simulink model "EMSLEVEL1"  (R2026a)
settings: Solver=FixedStepDiscrete  StopTime=86400  FixedStep=60
InitFcn:
  | params_ems;
  | cap = p.invACDC(p.P_lim);
values from neighbouring files (symbols this model uses):
  p = evalin('base', 'p')    [make_figures.m]    (also in params_ems.m = struct())
undefined symbols (not defined in the file or in its folder): DiscIntNeverNeededParam
settings Model: Creator=Kratos  LastModifiedBy=Kratos

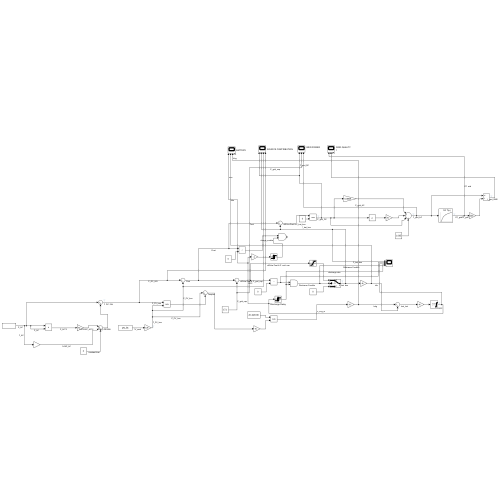
[thumbnail: Simulink's stored preview of the top-level diagram]
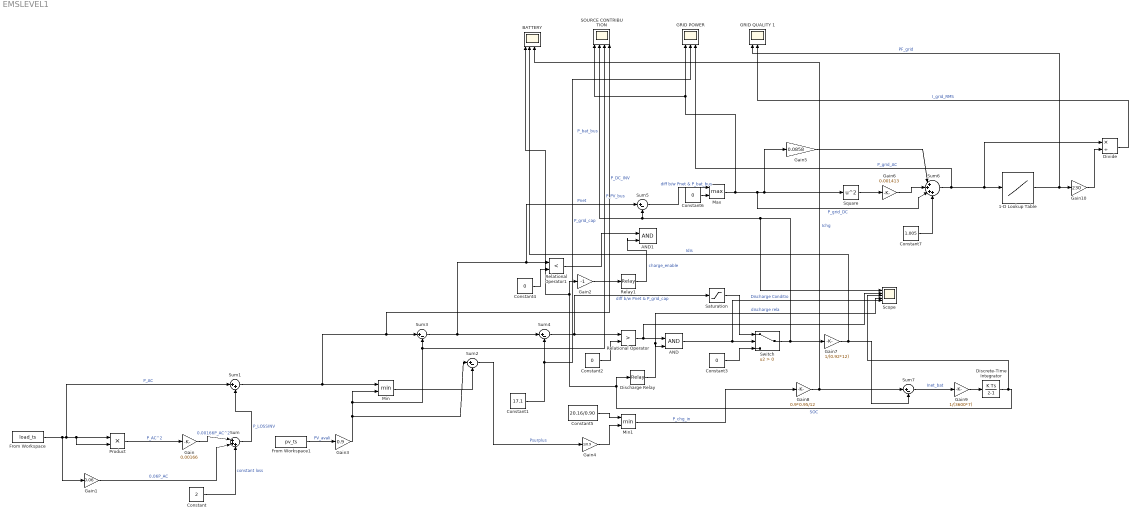
== system EMSLEVEL1 ==
  1-D Lookup Table : Lookup_n-D  NumberOfTableDimensions=1  BreakpointsForDimension1=[3.2 15.1 27.7 41.1 55.2]  Table=[0.308 0.364 0.386 0.399 0.408]  InternalRulePriority=Speed  RndMeth=Simplest
  AND : Logic  IconShape=distinctive  AllPortsSameDT=off  OutDataTypeStr=boolean
  AND1 : Logic  IconShape=distinctive  AllPortsSameDT=off  OutDataTypeStr=boolean
  BATTERY : Scope  NumInputPorts=4
      settings: ActiveDisplayYMinimum=0.046832535784003426  ActiveDisplayYMaximum=1.8408412036240656  DataLoggingVariableName=ScopeData2
  Constant : Constant  Value=2
  Constant1 : Constant  Value=17.1
  Constant{2..4,6} (4 alike) : Constant  Value=0
  Constant5 : Constant  Value=20.16/0.90
  Constant7 : Constant  Value=1.005
  Discharge Relay : Relay  OnSwitchValue=0.43  OffSwitchValue=0.40
  Discrete-Time Integrator : DiscreteIntegrator  InitialCondition=0.9  SampleTime=-1  LimitOutput=on  UpperSaturationLimit=1  LowerSaturationLimit=0  ICPrevOutput=DiscIntNeverNeededParam  ICPrevScaledInput=DiscIntNeverNeededParam
  Divide : Product  Inputs=*/
  From Workspace : FromWorkspace  VariableName=load_ts  SampleTime=60
  From Workspace1 : FromWorkspace  VariableName=pv_ts  SampleTime=60
  "GRID POWER " : Scope  NumInputPorts=3
      settings: ActiveDisplayYMinimum=6.4477565718978767  ActiveDisplayYMaximum=26.985680765987613
  GRID QUALITY 1 : Scope  NumInputPorts=3
      settings: ActiveDisplayYMinimum=-0.12702909452752709  ActiveDisplayYMaximum=0.73391197065675973  DataLoggingVariableName=ScopeData3
  Gain : Gain  Gain=0.00166
  Gain1 : Gain  Gain=0.06
  Gain10 : Gain  Gain=230
  Gain2 : Gain  Gain=-1
  Gain3 : Gain  Gain=0.9
  Gain4 : Gain  Gain=1/0.9
  Gain5 : Gain  Gain=0.0858
  Gain6 : Gain  Gain=0.001413
  Gain7 : Gain  Gain=1/(0.92*12)
  Gain8 : Gain  Gain=0.9*0.95/12
  Gain9 : Gain  Gain=1/(3600*7)
  Max : MinMax  Function=max  Inputs=2
  Min : MinMax  Inputs=2
  Min1 : MinMax  Inputs=2
  Product : Product
  Relational Operator : RelationalOperator  Operator=>  OutDataTypeStr=boolean  RndMeth=Simplest  InputSameDT=off
  Relational Operator1 : RelationalOperator  Operator=<  OutDataTypeStr=boolean  RndMeth=Simplest  InputSameDT=off
  Relay1 : Relay  OnSwitchValue=-0.87  OffSwitchValue=-0.90
  SOURCE CONTRIBUTION : Scope  NumInputPorts=4
      settings: ActiveDisplayYMinimum=28.409856286057689  ActiveDisplayYMaximum=45.225421172870654
  Saturation : Saturate  UpperLimit=30  LowerLimit=0
  Scope : Scope  NumInputPorts=5
      settings: ActiveDisplayYMinimum=-2.8927017969937969  ActiveDisplayYMaximum=27.832680981084884  DataLoggingVariableName=ScopeData4
  Square : Math  Operator=square
  Sum : Sum  Inputs=|+++
  Sum1 : Sum  Inputs=|++
  Sum{2..5,7} (5 alike) : Sum  Inputs=|+-
  Sum6 : Sum  Inputs=|++++
  Switch : Switch  Criteria=u2 > Threshold  SaturateOnIntegerOverflow=off  InputSameDT=off
  wires:
  From Workspace/1 -> Gain1/1, Sum1/1, Product/2, Product/1  "P_AC"
  Product/1 -> Gain/1  "P_AC^2"
  Gain/1 -> Sum/1  "0.00166P_AC^2"
  Gain1/1 -> Sum/2  "0.06P_AC"
  Constant/1 -> Sum/3  "constant loss"
  Sum/1 -> Sum1/2  "P_LOSSINV"
  Sum1/1 -> SOURCE CONTRIBUTION/4, Sum3/1, Min/1  "P_DC_INV"
  From Workspace1/1 -> Gain3/1  "PV_avali"
  Gain3/1 -> SOURCE CONTRIBUTION/3, Sum3/2, Min/2, Sum2/1  "P_PV_bus"
  Min/1 -> Sum2/2
  Sum2/1 -> Gain4/1  "Psurplus"
  Sum3/1 -> Sum5/1, Relational Operator1/1, Sum4/1  "Pnet"
  Gain2/1 -> Relay1/1
  Constant1/1 -> "GRID POWER "/2, Sum4/2  "P_grid_cap"
  Sum4/1 -> Saturation/1, Relational Operator/1  "diff b/w Pnet & P_grid_cap"
  Constant2/1 -> Relational Operator/2
  Relational Operator/1 -> Scope/2, AND/1
  Discharge Relay/1 -> Scope/4, AND/2  "discharge rela"
  AND/1 -> Scope/5, Switch/2  "Discharge Conditio"
  Saturation/1 -> Switch/1
  Constant3/1 -> Switch/3
  Switch/1 -> Scope/1, SOURCE CONTRIBUTION/2, Sum5/2, Gain7/1  "P_bat_bus"
  Constant4/1 -> Relational Operator1/2
  Relational Operator1/1 -> AND1/1
  Relay1/1 -> AND1/2  "charge_enable"
  Constant5/1 -> Min1/1
  Gain4/1 -> Min1/2
  Min1/1 -> Gain8/1  "P_chg_in"
  Sum5/1 -> Max/1  "diff b/w Pnet & P_bat_bus"
  Constant6/1 -> Max/2
  Max/1 -> Sum6/3, Gain5/1, Square/1, SOURCE CONTRIBUTION/1, "GRID POWER "/1  "P_grid_DC"
  Square/1 -> Gain6/1
  Gain5/1 -> Sum6/1
  Gain6/1 -> Sum6/2
  Constant7/1 -> Sum6/4
  Sum6/1 -> Divide/1, 1-D Lookup Table/1, "GRID POWER "/3  "P_grid_AC"
  Gain7/1 -> BATTERY/2, Sum7/2  "Idis"
  Gain8/1 -> Sum7/1, BATTERY/3  "Ichg"
  Sum7/1 -> Gain9/1  "Inet_bat"
  Gain9/1 -> Discrete-Time Integrator/1
  Discrete-Time Integrator/1 -> Scope/3, BATTERY/1, Gain2/1, Discharge Relay/1  "SOC"
  1-D Lookup Table/1 -> GRID QUALITY 1/1, Gain10/1  "PF_grid"
  Gain10/1 -> Divide/2
  Divide/1 -> GRID QUALITY 1/2  "I_grid_RMS"
